simulink model "ASP"  (R2022b)
settings: Solver=FixedStepDiscrete  StartTime=0.0  StopTime=inf  FixedStep=0.02  RelTol=1e-3
PreLoadFcn:
  | canMessageBusType;
  | canFDMessageBusType;
values from neighbouring files (symbols this model uses):
  ASP_HW_DEB_TIME = 100.0    [ASP.sldd]
  ASP_MODEL_CYCLE = 20.0    [ASP.sldd]
libraries: Mon3tr_Lib x1
PreSaveFcn:
  | filename = 'ASP';
  | dictionaryObj  = Simulink.data.dictionary.open([filename,'.sldd']);
  | saveChanges(dictionaryObj);
  | close(dictionaryObj);
  | disp([filename,'.sldd 已保存']);
settings Model: DataDictionary=ASP.sldd  Creator=Ligoo  LastModifiedBy=CENSORED
settings DataIOCC: SaveOutput=off  SignalLogging=off  DSMLogging=off  SaveTime=off  ReturnWorkspaceOutputs=off
settings OptimizationCC: DefaultParameterBehavior=Inlined  DefaultUnderspecifiedDataType=single  EnableMemcpy=off  ActiveStateOutputEnumStorageType=uint16  ZeroExternalMemoryAtStartup=off  ZeroInternalMemoryAtStartup=off  NoFixptDivByZeroProtection=on  EfficientFloat2IntCast=on  LifeSpan=Inf  MaxStackSize=200  OptimizeBlockOrder=speed  DifferentSizesBufferReuse=on  EfficientTunableParamExpr=on
settings DebuggingCC: SignalInfNanChecking=error  SignalRangeChecking=warning  AlgebraicLoopMsg=error  MergeDetectMultiDrivingBlocksExec=none  TasksWithSamePriorityMsg=error  IntegerOverflowMsg=error  UnconnectedInputMsg=error  UnconnectedOutputMsg=error  UnconnectedLineMsg=error  UniqueDataStoreMsg=warning  ModelReferenceIOMsg=error  ModelReferenceVersionMismatchMessage=error  StateNameClashWarn=warning  SFUnexpectedBacktrackingDiag=warning  SFNoUnconditionalDefaultTransitionDiag=warning  SFUndirectedBroadcastEventsDiag=error  IntegerSaturationMsg=error
settings HardwareCC: ProdBitPerPointer=32  ProdBitPerSizeT=32  ProdBitPerPtrDiffT=32  ProdLargestAtomicInteger=Long  ProdWordSize=32  ProdLongLongMode=on  ProdHWDeviceType=ARM Compatible->ARM 7
settings ModelReferenceCC: EnableRefExpFcnMdlSchedulingChecks=on
settings SFSimCC: MATLABDynamicMemAlloc=off
settings RTWCC: Description=Embedded Coder  SystemTargetFile=ert.tlc  GenCodeOnly=on  TemplateMakefile=ert_default_tmf  PostCodeGenCommand=FileCopy ASP  GenerateReport=on  RTWUseSimCustomCode=on  Toolchain=LCC-win64 v2.4.1 | gmake (64-bit Windows)  IncludeHyperlinkInReport=on  LaunchReport=on  GenerateTraceInfo=on  GenerateTraceReport=on  GenerateTraceReportSl=on  GenerateTraceReportSf=on  GenerateTraceReportEml=on
settings CodeAppCC: ForceParamTrailComments=on  IgnoreCustomStorageClasses=off  OperatorAnnotations=on  SimulinkDataObjDesc=on  SFDataObjDesc=on  MATLABFcnDesc=on  CustomSymbolStrUtil=$R$N$C  InsertBlockDesc=on  MATLABSourceComments=on
settings ERTTargetCC: MultiwordLength=2048  ConcurrentExecutionCompliant=off  IncludeMdlTerminateFcn=off  SuppressErrorStatus=on  SupportAbsoluteTime=off  SupportNonFinite=off  SupportComplex=off  ModelStepFunctionPrototypeControlCompliant=off  CPPClassGenCompliant=off  ArrayLayout=Row-major  GenerateASAP2=on  InlinedParameterPlacement=NonHierarchical  ERTCustomFileTemplate=example_file_process.tlc
settings ConfigComp: CovSaveCumulativeToWorkspaceVar=on  CovSaveSingleToWorkspaceVar=on  CovExternalEMLEnable=off  DVTestSuiteOptimization=CombinedObjectives (Nonlinear Extended)  DVDetectActiveLogic=on  DVModelReferenceHarness=on  DVHarnessSource=Signal Editor

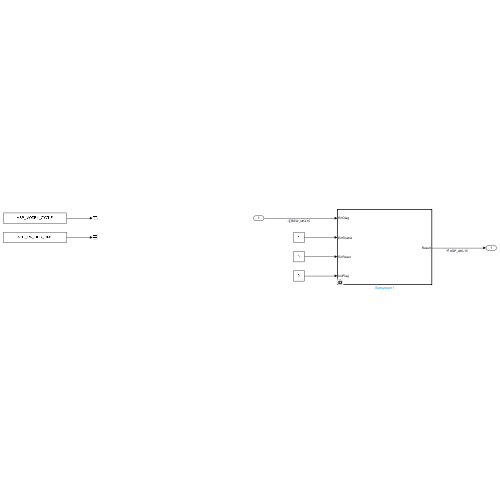
[thumbnail: Simulink's stored preview of the top-level diagram]
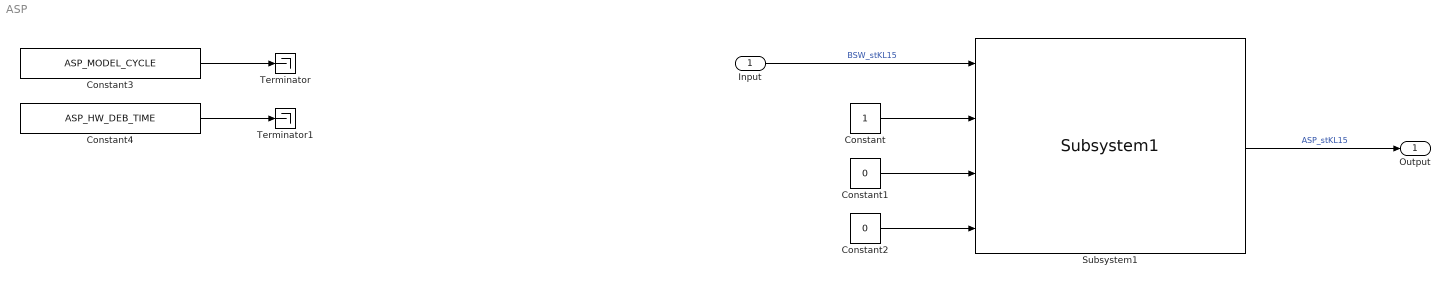
== system ASP ==
  Input : Inport
  Constant : Constant  OutDataTypeStr=uint8
  Constant1 : Constant  Value=0  OutDataTypeStr=uint8
  Constant2 : Constant  Value=0  OutDataTypeStr=uint8
  Constant3 : Constant  Value=ASP_MODEL_CYCLE
  Constant4 : Constant  Value=ASP_HW_DEB_TIME
  Subsystem1 : Mon3tr_Lib/Subsystem1  Model_Cycle=ASP_MODEL_CYCLE  DiagEnable=uint8(1)  DiagDealTime=ASP_HW_DEB_TIME  DiagHealTime=ASP_HW_DEB_TIME  DiagDealTimeInit=uint32(0)  DiagHealType=uint8(0)
  Terminator : Terminator
  Terminator1 : Terminator
  Output : Outport
  wires:
  Input/1 -> Subsystem1/1  "BSW_stKL15"
  Constant/1 -> Subsystem1/2
  Constant1/1 -> Subsystem1/3
  Constant2/1 -> Subsystem1/4
  Subsystem1/1 -> Output/1  "ASP_stKL15"
  Constant3/1 -> Terminator/1
  Constant4/1 -> Terminator1/1
